simulink model "dc_motor_test"  (R2026a)
settings: Solver=VariableStepAuto  StopTime=10
InitFcn:
  | init_motor;
undefined symbols (not defined in the file or in its folder): motor
settings Model: Creator=seman  LastModifiedBy=seman

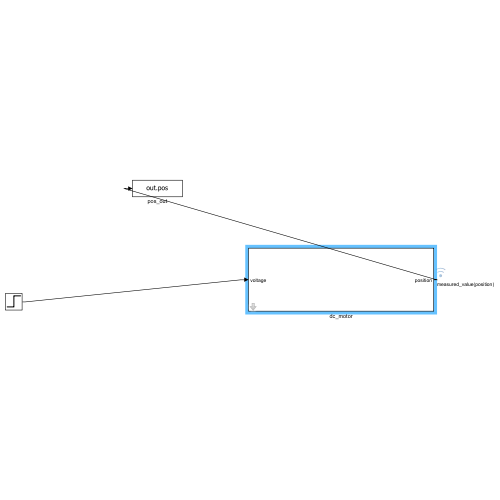
[thumbnail: Simulink's stored preview of the top-level diagram]
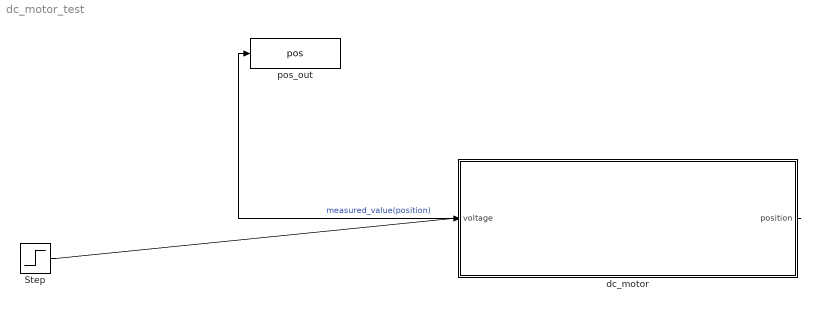
== system dc_motor_test ==
  Step : Step  Time=0  SampleTime=0
  dc_motor : Subsystem  InitFcn=""  mask{J=motor.J, B=motor.B, KT=motor.KT, R=motor.R, L=motor.L, KB=motor.KB}
      mask prompts: J "J(KG*M^2)"; B "B(Nm/rad)"; KT "NM/AMPER"; R "R(OHM)"; L "L(H)"; KB "KB(VS/rad)"
  pos_out : ToWorkspace  VariableName=pos  SaveFormat=Timeseries  SampleTime=-1
  wires:
  Step/1 -> dc_motor/1(voltage)
  dc_motor/1(position) -> pos_out/1  "measured_value(position)"

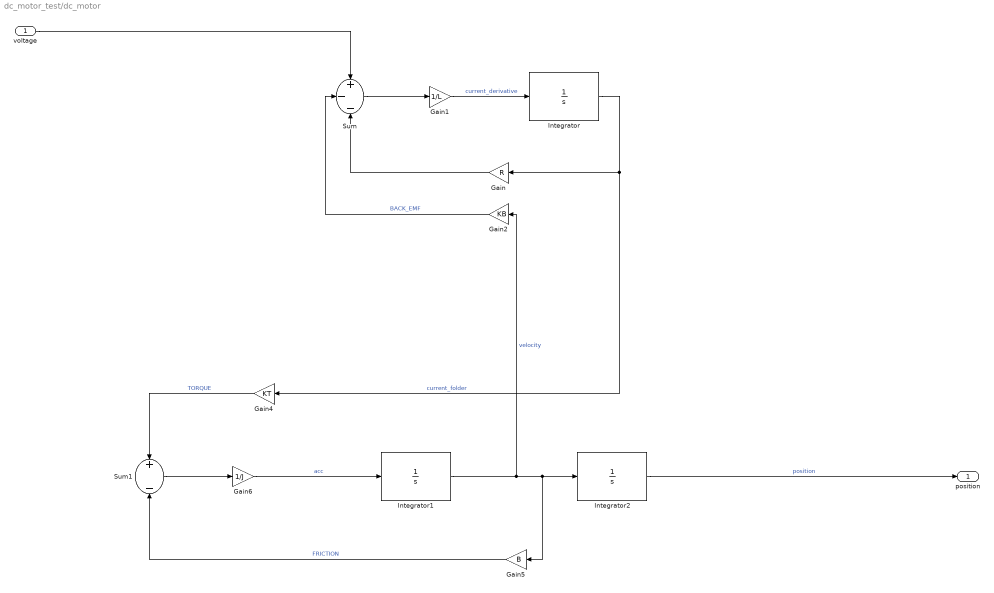
== system dc_motor_test/dc_motor ==
  voltage : Inport
  Gain : Gain  Gain=R
  Gain1 : Gain  Gain=1/L
  Gain2 : Gain  Gain=KB
  Gain4 : Gain  Gain=KT
  Gain5 : Gain  Gain=B
  Gain6 : Gain  Gain=1/J
  Integrator : Integrator
  Integrator1 : Integrator
  Integrator2 : Integrator
  Sum : Sum  Inputs=+--
  Sum1 : Sum  Inputs=+-
  position : Outport
  wires:
  voltage/1 -> Sum/1
  Integrator2/1 -> position/1  "position"
  Gain5/1 -> Sum1/2  "FRICTION"
  Sum1/1 -> Gain6/1
  Gain1/1 -> Integrator/1  "current_derivative"
  Sum/1 -> Gain1/1
  Gain/1 -> Sum/3
  Integrator/1 -> Gain/1, Gain4/1  "current_folder"
  Gain4/1 -> Sum1/1  "TORQUE"
  Gain2/1 -> Sum/2  "BACK_EMF"
  Integrator1/1 -> Gain5/1, Integrator2/1, Gain2/1  "velocity"
  Gain6/1 -> Integrator1/1  "acc"
